simulink model "PreLab1 + 2"  (R2021a)
settings: Solver=VariableStepAuto  StartTime=0.0  StopTime=5  FixedStep=1/40000  MaxStep=0.000001  RelTol=1e-9
libraries: dsparch4 x6
settings Model: Creator=Mataya  LastModifiedBy=Mataya

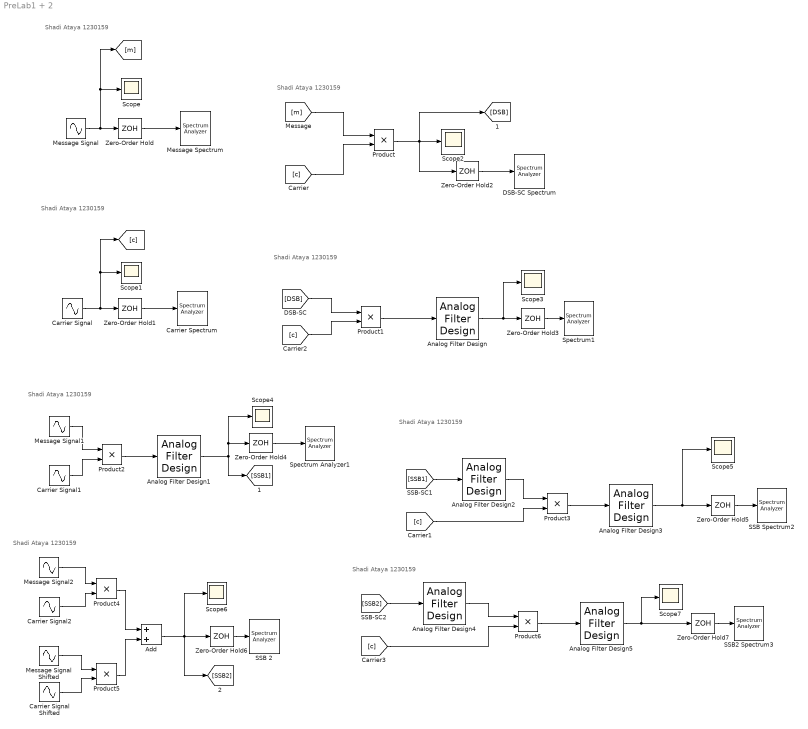
== system PreLab1 + 2 ==
  note: Shadi Ataya 1230159
  note: Shadi Ataya 1230159
  note: Shadi Ataya 1230159
  note: Shadi Ataya 1230159
  note: Shadi Ataya 1230159
  note: Shadi Ataya 1230159
  note: Shadi Ataya 1230159
  note: Shadi Ataya 1230159
  " Spectrum1" : SpectrumAnalyzer
  Add : Sum
  Analog Filter Design : dsparch4/Analog Filter Design  method=Butterworth  filttype=Lowpass  N=4  Wlo=1000*2*pi  Whi=80  Rp=2  Rs=40
  Analog Filter Design1 : dsparch4/Analog Filter Design  method=Butterworth  filttype=Bandpass  N=2  Wlo=13800*2*pi  Whi=14200*2*pi  Rp=2  Rs=40
  Analog Filter Design2 : dsparch4/Analog Filter Design  method=Butterworth  filttype=Bandpass  N=2  Wlo=13000*2*pi  Whi=14500*2*pi  Rp=2  Rs=40
  Analog Filter Design3 : dsparch4/Analog Filter Design  method=Butterworth  filttype=Lowpass  N=4  Wlo=1000*2*pi  Whi=80  Rp=2  Rs=40
  Analog Filter Design4 : dsparch4/Analog Filter Design  method=Butterworth  filttype=Bandpass  N=2  Wlo=13000*2*pi  Whi=14500*2*pi  Rp=2  Rs=40
  Analog Filter Design5 : dsparch4/Analog Filter Design  method=Butterworth  filttype=Lowpass  N=4  Wlo=1000*2*pi  Whi=80  Rp=2  Rs=40
  Carrier Spectrum : SpectrumAnalyzer
  Carrier Signal : Sin  Frequency=15000*2*pi  Phase=pi/2  SampleTime=0
  Carrier Signal Shifted : Sin  Frequency=15000*2*pi  SampleTime=0
  Carrier Signal1 : Sin  Frequency=15000*2*pi  Phase=pi/2  SampleTime=0
  Carrier Signal2 : Sin  Frequency=15000*2*pi  Phase=pi/2  SampleTime=0
  DSB-SC Spectrum : SpectrumAnalyzer
  Message Spectrum : SpectrumAnalyzer
  Message Signal : Sin  Amplitude=0.85  Frequency=1000*2*pi  Phase=pi/2  SampleTime=0
  Message Signal Shifted : Sin  Amplitude=0.85  Frequency=1000*2*pi  SampleTime=0
  Message Signal1 : Sin  Amplitude=0.85  Frequency=1000*2*pi  Phase=pi/2  SampleTime=0
  Message Signal2 : Sin  Amplitude=0.85  Frequency=1000*2*pi  Phase=pi/2  SampleTime=0
  Product{,1..6} (7 alike) : Product
  SSB Spectrum2 : SpectrumAnalyzer
  SSB 2 : SpectrumAnalyzer
  SSB2 Spectrum3 : SpectrumAnalyzer
  Scope{,1..7} (8 alike) : Scope
  Spectrum Analyzer1 : SpectrumAnalyzer
  Zero-Order Hold{,1..7} (8 alike) : ZeroOrderHold  SampleTime=1/40000
  wires:
  Message Signal/1 -> Zero-Order Hold/1, [m], Scope/1
  Zero-Order Hold/1 -> Message Spectrum/1
  Zero-Order Hold1/1 -> Carrier Spectrum/1
  Carrier Signal/1 -> [c], Scope1/1, Zero-Order Hold1/1
  Zero-Order Hold2/1 -> DSB-SC Spectrum/1
  Product/1 -> Zero-Order Hold2/1, [DSB], Scope2/1
  [c] -> Product/2
  [m] -> Product/1
  Analog Filter Design/1 -> Scope3/1, Zero-Order Hold3/1
  Product1/1 -> Analog Filter Design/1
  [DSB] -> Product1/1
  [c] -> Product1/2
  Zero-Order Hold3/1 -> " Spectrum1"/1
  Carrier Signal1/1 -> Product2/2
  Zero-Order Hold4/1 -> Spectrum Analyzer1/1
  Product2/1 -> Analog Filter Design1/1
  Message Signal1/1 -> Product2/1
  Analog Filter Design1/1 -> Scope4/1, Zero-Order Hold4/1, [SSB1]
  [SSB1] -> Analog Filter Design2/1
  Product3/1 -> Analog Filter Design3/1
  Zero-Order Hold5/1 -> SSB Spectrum2/1
  [c] -> Product3/2
  Analog Filter Design3/1 -> Scope5/1, Zero-Order Hold5/1
  Analog Filter Design2/1 -> Product3/1
  Carrier Signal Shifted/1 -> Product5/2
  Zero-Order Hold6/1 -> SSB 2/1
  Message Signal Shifted/1 -> Product5/1
  Carrier Signal2/1 -> Product4/2
  Add/1 -> Scope6/1, [SSB2], Zero-Order Hold6/1
  Product4/1 -> Add/1
  Product5/1 -> Add/2
  Message Signal2/1 -> Product4/1
  [SSB2] -> Analog Filter Design4/1
  [c] -> Product6/2
  Analog Filter Design5/1 -> Zero-Order Hold7/1, Scope7/1
  Zero-Order Hold7/1 -> SSB2 Spectrum3/1
  Analog Filter Design4/1 -> Product6/1
  Product6/1 -> Analog Filter Design5/1
